simulink model "acc_closed_loop"  (R2026b)
settings: Solver=ode3  StopTime=60  FixedStep=0.005
undefined symbols (not defined in the file or in its folder): acc_plant_params, scn_act_valid, scn_mass_prior, scn_pitch_known
settings Model: Creator=kikiw  LastModifiedBy=kikiw
settings SolverCC: AutoInsertRateTranBlk=on
settings DataIOCC: SignalLogging=off

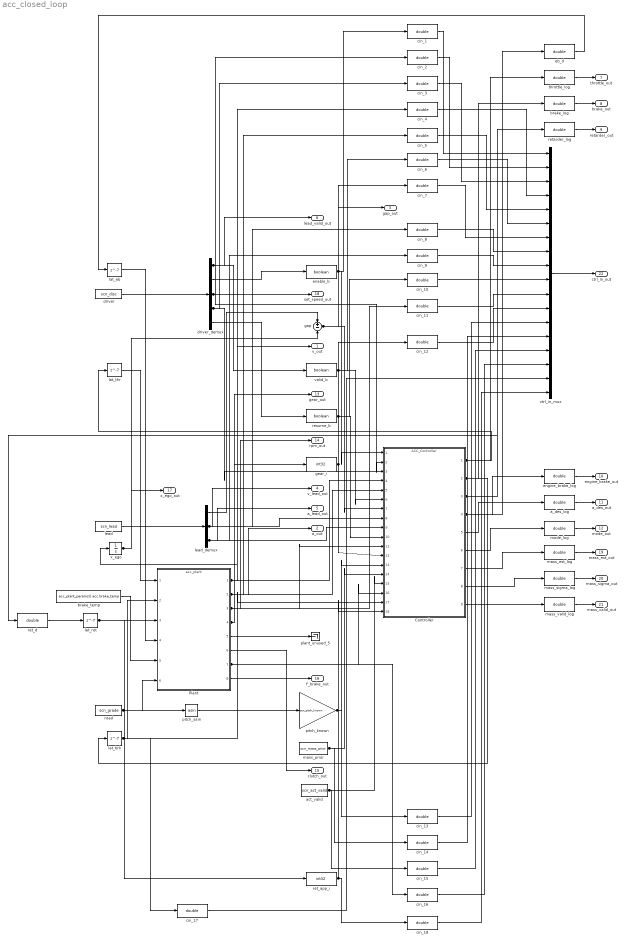
== system acc_closed_loop ==
  Controller : ModelReference  ModelNameDialog=ACC_Controller  SimulationMode=Normal  ModelReferenceVersion=1.1
  Plant : ModelReference  ModelNameDialog=acc_plant  SimulationMode=Normal  ModelReferenceVersion=1.1
  a_des_log : DataTypeConversion  OutDataTypeStr=double  SaturateOnIntegerOverflow=off  RndMeth=Floor
  act_valid : Constant  Value=scn_act_valid  OutDataTypeStr=boolean
  brake_log : DataTypeConversion  OutDataTypeStr=double  SaturateOnIntegerOverflow=off  RndMeth=Floor
  brake_temp : Constant  Value=acc_plant_params().acc.brake_temp
  cin_{1..18} (18 alike) : DataTypeConversion  OutDataTypeStr=double  SaturateOnIntegerOverflow=off  RndMeth=Floor
  ctrl_in_mux : Mux  Inputs=18
  driver : FromWorkspace  VariableName=scn_disc  SampleTime=0.05  Interpolate=off  OutputAfterFinalValue=Holding final value
  driver_demux : Demux  Outputs=5
  eb_d : DataTypeConversion  OutDataTypeStr=double  SaturateOnIntegerOverflow=off  RndMeth=Floor
  enable_b : DataTypeConversion  OutDataTypeStr=boolean  SaturateOnIntegerOverflow=off  RndMeth=Floor
  engine_brake_log : DataTypeConversion  OutDataTypeStr=double  SaturateOnIntegerOverflow=off  RndMeth=Floor
  gap : Sum  Inputs=+-
  gear_i : DataTypeConversion  OutDataTypeStr=int32  SaturateOnIntegerOverflow=off  RndMeth=Floor
  lat_brk : Delay  DelayLength=7  InitialCondition=0  SampleTime=0.005
  lat_eb : Delay  DelayLength=7  InitialCondition=0  SampleTime=0.005
  lat_ret : Delay  DelayLength=7  InitialCondition=0  SampleTime=0.005
  lat_thr : Delay  DelayLength=7  InitialCondition=0  SampleTime=0.005
  lead : FromWorkspace  VariableName=scn_lead  OutputAfterFinalValue=Holding final value
  lead_demux : Demux  Outputs=3
  mass_est_log : DataTypeConversion  OutDataTypeStr=double  SaturateOnIntegerOverflow=off  RndMeth=Floor
  mass_prior : Constant  Value=scn_mass_prior
  mass_sigma_log : DataTypeConversion  OutDataTypeStr=double  SaturateOnIntegerOverflow=off  RndMeth=Floor
  mass_valid_log : DataTypeConversion  OutDataTypeStr=double  SaturateOnIntegerOverflow=off  RndMeth=Floor
  mode_log : DataTypeConversion  OutDataTypeStr=double  SaturateOnIntegerOverflow=off  RndMeth=Floor
  pitch_asin : Trigonometry  Operator=asin
  pitch_known : Gain  Gain=scn_pitch_known
  plant_unused_5 : Terminator
  resume_b : DataTypeConversion  OutDataTypeStr=boolean  SaturateOnIntegerOverflow=off  RndMeth=Floor
  ret_app_i : DataTypeConversion  OutDataTypeStr=int32  SaturateOnIntegerOverflow=off  RndMeth=Floor
  ret_d : DataTypeConversion  OutDataTypeStr=double  SaturateOnIntegerOverflow=off  RndMeth=Floor
  retarder_log : DataTypeConversion  OutDataTypeStr=double  SaturateOnIntegerOverflow=off  RndMeth=Floor
  road : FromWorkspace  VariableName=scn_grade  OutputAfterFinalValue=Holding final value
  throttle_log : DataTypeConversion  OutDataTypeStr=double  SaturateOnIntegerOverflow=off  RndMeth=Floor
  valid_b : DataTypeConversion  OutDataTypeStr=boolean  SaturateOnIntegerOverflow=off  RndMeth=Floor
  x_ego : Integrator
  v_out : Outport
  a_out : Outport  Port=2
  gap_out : Outport  Port=3
  v_lead_out : Outport  Port=4
  a_lead_out : Outport  Port=5
  lead_valid_out : Outport  Port=6
  throttle_out : Outport  Port=7
  brake_out : Outport  Port=8
  retarder_out : Outport  Port=9
  engine_brake_out : Outport  Port=10
  a_des_out : Outport  Port=11
  mode_out : Outport  Port=12
  gear_out : Outport  Port=13
  rpm_out : Outport  Port=14
  clutch_out : Outport  Port=15
  F_brake_out : Outport  Port=16
  x_ego_out : Outport  Port=17
  set_speed_out : Outport  Port=18
  mass_est_out : Outport  Port=19
  mass_sigma_out : Outport  Port=20
  mass_valid_out : Outport  Port=21
  ctrl_in_out : Outport  Port=22
  wires:
  brake_temp/1 -> Plant/5
  cin_4/1 -> ctrl_in_mux/4
  pitch_known/1 -> Controller/13, cin_13/1
  eb_d/1 -> lat_eb/1
  lat_thr/1 -> Plant/1
  cin_1/1 -> ctrl_in_mux/1
  ret_d/1 -> lat_ret/1
  Plant/7 -> cin_16/1, Controller/16
  lat_ret/1 -> Plant/3, ret_app_i/1
  Controller/5 -> a_des_log/1
  driver/1 -> driver_demux/1
  Controller/4 -> eb_d/1, engine_brake_log/1
  lat_eb/1 -> Plant/4
  enable_b/1 -> Controller/1, cin_1/1
  Controller/2 -> lat_brk/1, brake_log/1
  lead_demux/2 -> Controller/8, cin_8/1, v_lead_out/1
  lead/1 -> lead_demux/1
  act_valid/1 -> Controller/15, cin_15/1
  x_ego/1 -> gap/2, x_ego_out/1
  road/1 -> Plant/6, pitch_asin/1
  cin_5/1 -> ctrl_in_mux/5
  lat_brk/1 -> Controller/17, cin_17/1, Plant/2
  cin_2/1 -> ctrl_in_mux/2
  driver_demux/1 -> valid_b/1, lead_valid_out/1
  driver_demux/2 -> enable_b/1
  driver_demux/3 -> cin_2/1, Controller/2, set_speed_out/1
  driver_demux/4 -> Controller/3, cin_3/1
  driver_demux/5 -> resume_b/1
  lead_demux/1 -> gap/1
  Controller/1 -> throttle_log/1, lat_thr/1
  lead_demux/3 -> Controller/9, cin_9/1, a_lead_out/1
  cin_18/1 -> ctrl_in_mux/18
  Plant/5 -> plant_unused_5/1
  cin_15/1 -> ctrl_in_mux/15
  Plant/1 -> x_ego/1, cin_4/1, v_out/1, Controller/4
  cin_11/1 -> ctrl_in_mux/11
  cin_8/1 -> ctrl_in_mux/8
  cin_12/1 -> ctrl_in_mux/12
  Plant/2 -> Controller/5, cin_5/1, a_out/1
  cin_13/1 -> ctrl_in_mux/13
  Plant/3 -> Controller/11, rpm_out/1, cin_11/1
  cin_14/1 -> ctrl_in_mux/14
  Plant/4 -> gear_i/1, gear_out/1
  cin_10/1 -> ctrl_in_mux/10
  Plant/6 -> clutch_out/1
  Plant/8 -> F_brake_out/1
  pitch_asin/1 -> pitch_known/1
  cin_9/1 -> ctrl_in_mux/9
  cin_17/1 -> ctrl_in_mux/17
  cin_6/1 -> ctrl_in_mux/6
  valid_b/1 -> Controller/6, cin_6/1
  gap/1 -> gap_out/1, cin_7/1, Controller/7
  resume_b/1 -> Controller/10, cin_10/1
  gear_i/1 -> cin_12/1, Controller/12
  mass_prior/1 -> Controller/14, cin_14/1
  ret_app_i/1 -> Controller/18, cin_18/1
  cin_3/1 -> ctrl_in_mux/3
  cin_7/1 -> ctrl_in_mux/7
  Controller/3 -> ret_d/1, retarder_log/1
  Controller/6 -> mode_log/1
  Controller/7 -> mass_est_log/1
  Controller/8 -> mass_sigma_log/1
  Controller/9 -> mass_valid_log/1
  cin_16/1 -> ctrl_in_mux/16
  throttle_log/1 -> throttle_out/1
  brake_log/1 -> brake_out/1
  retarder_log/1 -> retarder_out/1
  ctrl_in_mux/1 -> ctrl_in_out/1
  engine_brake_log/1 -> engine_brake_out/1
  a_des_log/1 -> a_des_out/1
  mode_log/1 -> mode_out/1
  mass_est_log/1 -> mass_est_out/1
  mass_sigma_log/1 -> mass_sigma_out/1
  mass_valid_log/1 -> mass_valid_out/1
